simulink model "powersystem"  (R2026a)
settings: Solver=VariableStepAuto  StopTime=0.2
libraries: ee_lib x4, fl_lib x1, nesl_utility x1
settings Model: Creator=santr  LastModifiedBy=santr

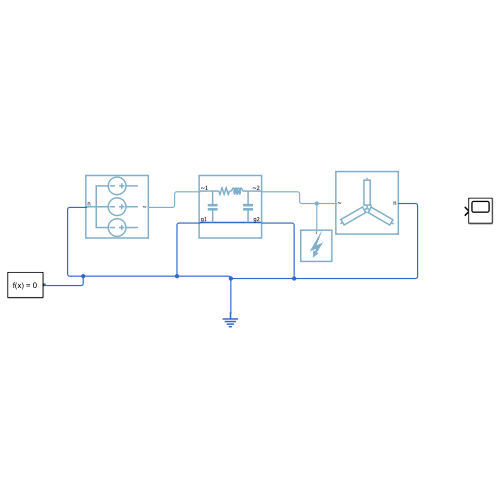
[thumbnail: Simulink's stored preview of the top-level diagram]
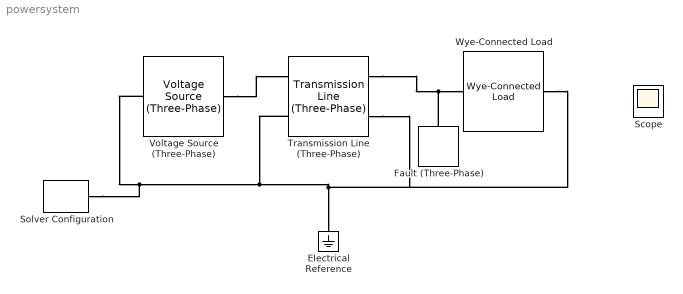
== system powersystem ==
  Electrical Reference : fl_lib/Electrical/Electrical Elements/Electrical Reference
  Fault (Three-Phase) : ee_lib/Utilities/Fault (Three-Phase)  port_option=ee.enum.threePhasePort.composite  fault_type_option=ee.enum.fault_type_option.ag  R_pn_fault=1e-3 Ohm  R_ng_fault=1e-3 Ohm  exposemeasurement=ee.enum.exposemeasurement.hidden  enable_external_fault=ee.enum.external_fault.hidden  fault_threshold=0.5  fault_condition=ee.enum.fault_condition.fgt  fault_resettable=ee.enum.enable.no  enable_temporal_fault=ee.enum.enable.no  fault_start_time=1 s  fault_duration=0.1 s  G_parasitic=1e-4 1/Ohm  I_specify=off  I_priority=None  I=[0, 0, 0] A  I_nominal_specify=off  I_nominal_value=1  I_nominal_unit=A  i_ng_specify=off  i_ng_priority=None  i_ng=0 A  i_ng_nominal_specify=off  i_ng_nominal_value=1  i_ng_nominal_unit=A
  Scope : Scope
  Solver Configuration : nesl_utility/Solver Configuration  PhysicalDomain=network_engine_domain  SubClassName=solver  LeftPortType=input  RightPortType=generic  Tones=[]  Harmonics=[]  SimulateNoise=off  Profile=off  UseLocalSampling=off  EnableSwitchedLinearOptims=on  FrequencyDomain=off  UseCCode=off  RelTol=0.001  AbsTol=0.001  MinStep=1e-09  ToWorkspace=off  RevertToSquareIcSolve=off  NumHomotopyIterations=100  PhasorMode=off  PhasorModeNumHarmonics=1  ConsistencySolver=NEWTON_XTOL_AFTER_FTOL  CanonicalOrdering=CANONICAL  OptimizeIntermediates=OPTIMIZED  IndexReductionMethod=DerivativeReplacement  DoDC=off  ResidualTolerance=1e-09  ConsistencyTolSource=GLOBAL  ConsistencyAbsTol=0.001  ConsistencyRelTol=0.001  ConsistencyTolFactor=0.001  UseLocalSolver=off  LocalSolverChoice=NE_BACKWARD_EULER_ADVANCER  ResolveIndetEquations=on  FunctionEvalNumThread=1  LocalSolverSampleTime=0.001  DoFixedCost=off  MaxNonlinIter=3  MaxModeIter=2  ComputeImpulses=off  ImpulseIterations=2  LinearAlgebra=auto  LinearAlgebraNumThread=0  EquationFormulation=NE_TIME_EF  DelaysMemoryBudget=1024  AutomaticFiltering=on  FilteringTimeConstant=0.001  PartitionStorageMethod=AS_NEEDED  PartitionMemoryBudget=1024  PartitionMethod=ROBUST  MultibodyUseLocalSolver=off  MultibodyLocalSolverChoice=ODE1  MultibodyLocalSolverSampleTime=0.001
  Transmission Line (Three-Phase) : ee_lib/Passive/Lines/Transmission Line (Three-Phase)  port_option=ee.enum.threePhasePort.composite  length=50 km  freq=50 Hz  prm=ee.enum.lines.parameterization3ph.physicalLineParam  R=0.2 Ohm/km  Rm=0 Ohm/km  L=1 H/km  M=0.1 mH/km  Cl=0.5 uF/km  Cg=10 nF/km  Rpos=0.01 Ohm/km  Rzero=0.04 Ohm/km  Lpos=0.4 mH/km  Lzero=0.7 mH/km  Cpos=1 uF/km  Czero=0.1 uF/km  ModelTwoSections=ee.enum.enable.no  N=1  InterfacePosition=0.5 km  N1sec=1  N2sec=1  Access_ground=ee.enum.enable.no  R_parasitic=1e-6 Ohm  G_parasitic=1e-6 1/Ohm
  Voltage Source (Three-Phase) : ee_lib/Sources/Voltage Source (Three-Phase)  vline_rms=11 kV  shift=0 deg  freq=50 Hz  impedance_option=1  SShortCircuit=1e6 A*V  XR=15  R=0.01 Ohm  L=3.97e-4 H  harmonic_option=0  harmonic_orders=[5, 7, 11, 13]  harmonic_ratios=[.1, .1, .1, .1]  G_parasitic=0 1/Ohm  I_specify=off  I_priority=None  I=[0, 0, 0] A  I_nominal_specify=off  I_nominal_value=1  I_nominal_unit=A
  Wye-Connected Load : ee_lib/Passive/RLC Assemblies/Wye-Connected Load  port_option=ee.enum.threePhasePort.composite  parameterization=ee.enum.rlc.parameterization.ratedpower  component_structure=ee.enum.rlc.structure.R  component_structure_PQ=ee.enum.rlc.structure.SeriesRL  R=1 Ohm  L=1e-3 H  C=1e-6 F  VRated=11 kV  FRated=50 Hz  P=1 mW  Qpos=5e5 V*A  Qneg=-1e2 A*V  R_parasitic=0 Ohm  G_parasitic=0 1/Ohm  R_parasitic_PQ=0 Ohm  G_parasitic_PQ=0 1/Ohm  Vmag0=24e3 V  Vang0=0 deg  Freq0=60 Hz  IL_specify=off  IL_priority=High  IL=[0, 0, 0] A  IL_nominal_specify=off  IL_nominal_value=1  IL_nominal_unit=A  VC_specify=off  VC_priority=High  VC=[0, 0, 0] V  VC_nominal_specify=off  VC_nominal_value=1  VC_nominal_unit=V
  connections:
  Voltage Source (Three-Phase)/RConn1 -- Transmission Line (Three-Phase)/LConn1
  Transmission Line (Three-Phase)/RConn1 -- Fault (Three-Phase)/LConn1 -- Wye-Connected Load/LConn1
  Voltage Source (Three-Phase)/LConn1 -- Solver Configuration/RConn1 -- Transmission Line (Three-Phase)/LConn2 -- Transmission Line (Three-Phase)/RConn2 -- Wye-Connected Load/RConn1 -- Electrical Reference/LConn1
